simulink model "simautod1"  (Simulink 3.00)
settings: Solver=ode45  StartTime=0.0  StopTime=10  MaxStep=.01  RelTol=1e-6  AbsTol=1e-6
values from neighbouring files (symbols this model uses):
  STATEInit = [0, 1.0, 0, 0]    [objauto2.m]
  TIMEdis = 0.05    [objauto2.m]
undefined symbols (not defined in the file or in its folder): Adis, Bdis, Cdis, Ddis, DenContr, NumContr
settings Model: SaveTime=off  SaveOutput=off  LastModifiedBy=pohlheim

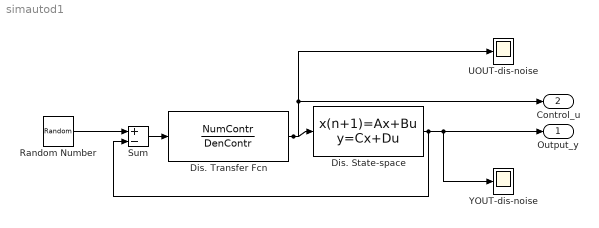
== system simautod1 ==
  Dis. State-space : DiscreteStateSpace  A=Adis  B=Bdis  C=Cdis  D=Ddis  X0=STATEInit  SampleTime=TIMEdis
  Dis. Transfer Fcn : DiscreteTransferFcn  Numerator=NumContr  Denominator=DenContr  SampleTime=TIMEdis
  Random Number : RandomNumber  Mean=0  Variance=0.001  Seed=12345  SampleTime=TIMEdis
  Sum : Sum  Inputs=+-  SaturateOnIntegerOverflow=on
  UOUT-dis-noise : Scope
      settings: TimeRange=11.000000  YMin=-0.2  YMax=0.2  SaveToWorkspace=off  SaveName=ScopeData  DataFormat=Matrix
  YOUT-dis-noise : Scope
      settings: TimeRange=11.000000  YMin=-1  YMax=1  SaveToWorkspace=off  SaveName=ScopeData  DataFormat=Matrix
  Output_y : Outport  Port=1
  Control_u : Outport  Port=2
  wires:
  Sum/1 -> Dis. Transfer Fcn/1
  Dis. State-space/1 -> Sum/2, YOUT-dis-noise/1, Output_y/1
  Dis. Transfer Fcn/1 -> Dis. State-space/1, UOUT-dis-noise/1, Control_u/1
  Random Number/1 -> Sum/1
